simulink model "Kamerastabilisierung"  (R2026a)
settings: Solver=ode4  StopTime=SIM.Tend  FixedStep=SIM.Ts
values from neighbouring files (symbols this model uses):
  GEL = par_gelenk(Z1)    [start_model.m]
  HOE = par_hoehe(SIM, rauschen = STUFE >= 3)    [start_model.m]
  MONT = par_montage()    [start_model.m]
  REG = par_regler(SIM, Z1, MONT)    [start_model.m]
  SEN = par_sensor(SIM, rauschen = STUFE >= 3)    [start_model.m]
  SIM = par_sim("vorn")    [start_model.m]
undefined symbols (not defined in the file or in its folder): Z1
settings Model: NumberOfSteps=2  Creator=johannes  LastModifiedBy=johannes

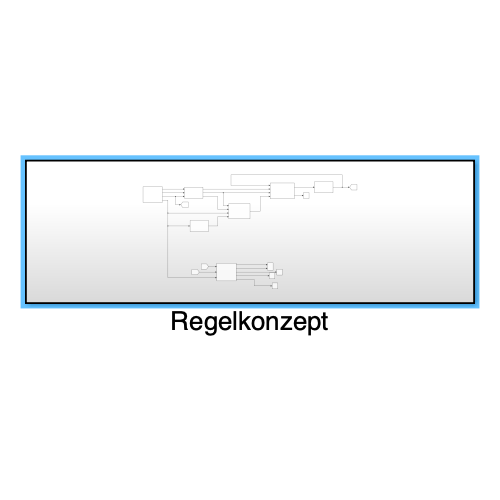
[thumbnail: Simulink's stored preview of the top-level diagram]
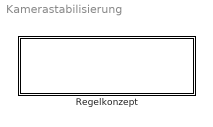
== system Kamerastabilisierung ==
  Regelkonzept : Subsystem

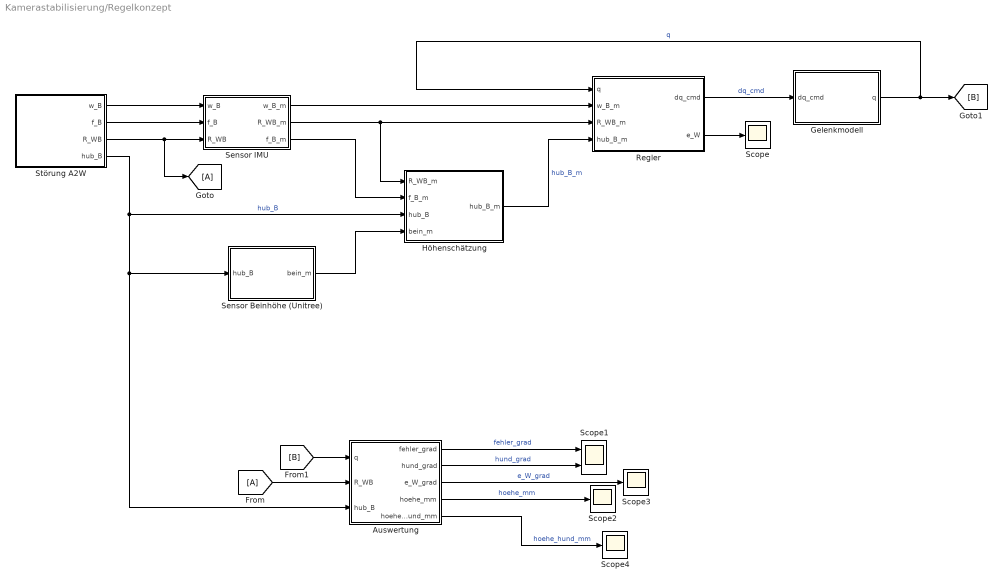
== system Kamerastabilisierung/Regelkonzept ==
  Auswertung : Subsystem
  From : From
  Gelenkmodell : Subsystem  Variant=on
  Goto : Goto
  Höhenschätzung : Subsystem  Variant=on
  Regler : Subsystem
  Scope{,2..4} (4 alike) : Scope
      Scope settings: ActiveDisplayYMinimum=-1  ActiveDisplayYMaximum=1  DataLoggingVariableName=ScopeData4
      Scope2 settings: ActiveDisplayYMinimum=-1  ActiveDisplayYMaximum=1
      Scope3 settings: ActiveDisplayYMinimum=-1  ActiveDisplayYMaximum=1  DataLoggingVariableName=ScopeData7
      Scope4 settings: ActiveDisplayYMinimum=-1  ActiveDisplayYMaximum=1  DataLoggingVariableName=ScopeData2
  Scope1 : Scope  NumInputPorts=2
      settings: ActiveDisplayYMinimum=-1  ActiveDisplayYMaximum=1
  Sensor Beinhöhe (Unitree) : Subsystem  Variant=on
  Sensor IMU : Subsystem  Variant=on
  Störung A2W : Subsystem
  wires:
  Störung A2W/3(R_WB) -> Goto/1, Sensor IMU/3(R_WB)
  Regler/2(e_W) -> Scope/1
  Auswertung/3(e_W_grad) -> Scope3/1  "e_W_grad"
  Auswertung/1(fehler_grad) -> Scope1/1  "fehler_grad"
  Auswertung/2(hund_grad) -> Scope1/2  "hund_grad"
  Störung A2W/1(w_B) -> Sensor IMU/1(w_B)
  Sensor IMU/1(w_B_m) -> Regler/2(w_B_m)
  Sensor IMU/2(R_WB_m) -> Regler/3(R_WB_m), Höhenschätzung/1(R_WB_m)
  Regler/1(dq_cmd) -> Gelenkmodell/1(dq_cmd)  "dq_cmd"
  Gelenkmodell/1(q) -> [B], Regler/1(q)  "q"
  Störung A2W/4(hub_B) -> Sensor Beinhöhe (Unitree)/1(hub_B), Auswertung/3(hub_B), Höhenschätzung/3(hub_B)  "hub_B"
  Auswertung/4(hoehe_mm) -> Scope2/1  "hoehe_mm"
  Auswertung/5(hoehe_hund_mm) -> Scope4/1  "hoehe_hund_mm"
  Störung A2W/2(f_B) -> Sensor IMU/2(f_B)
  Sensor IMU/3(f_B_m) -> Höhenschätzung/2(f_B_m)
  Höhenschätzung/1(hub_B_m) -> Regler/4(hub_B_m)  "hub_B_m"
  Sensor Beinhöhe (Unitree)/1(bein_m) -> Höhenschätzung/4(bein_m)
  From/1 -> Auswertung/2(R_WB)
  [B] -> Auswertung/1(q)

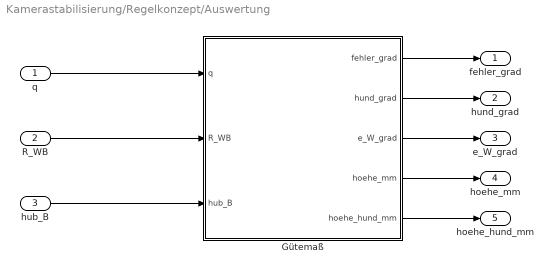
== system Kamerastabilisierung/Regelkonzept/Auswertung ==
  q : Inport
  R_WB : Inport  Port=2
  hub_B : Inport  Port=3
  Gütemaß : MATLAB Function  TreatAsAtomicUnit=on
  fehler_grad : Outport
  hund_grad : Outport  Port=2
  e_W_grad : Outport  Port=3
  hoehe_mm : Outport  Port=4
  hoehe_hund_mm : Outport  Port=5
  wires:
  Gütemaß/1(fehler_grad) -> fehler_grad/1
  Gütemaß/2(hund_grad) -> hund_grad/1
  Gütemaß/3(e_W_grad) -> e_W_grad/1
  hub_B/1 -> Gütemaß/3(hub_B)
  Gütemaß/4(hoehe_mm) -> hoehe_mm/1
  Gütemaß/5(hoehe_hund_mm) -> hoehe_hund_mm/1
  q/1 -> Gütemaß/1(q)
  R_WB/1 -> Gütemaß/2(R_WB)

== system Kamerastabilisierung/Regelkonzept/Gelenkmodell ==
  dq_cmd : Inport
  Ideal : Subsystem  VariantControl=STUFE == 1
  Realistisch : Subsystem  VariantControl=STUFE >= 2
  q : Outport

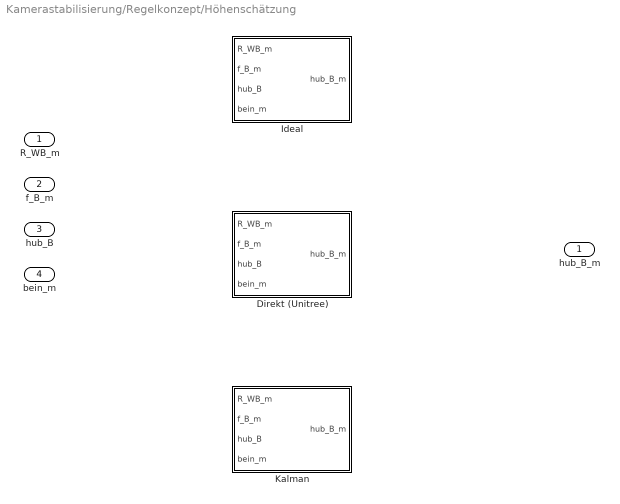
== system Kamerastabilisierung/Regelkonzept/Höhenschätzung ==
  R_WB_m : Inport
  f_B_m : Inport  Port=2
  hub_B : Inport  Port=3
  bein_m : Inport  Port=4
  Direkt (Unitree) : Subsystem  VariantControl=HOEHE_QUELLE == 2
  Ideal : Subsystem  VariantControl=HOEHE_QUELLE == 1
  Kalman : Subsystem  VariantControl=HOEHE_QUELLE == 3
  hub_B_m : Outport

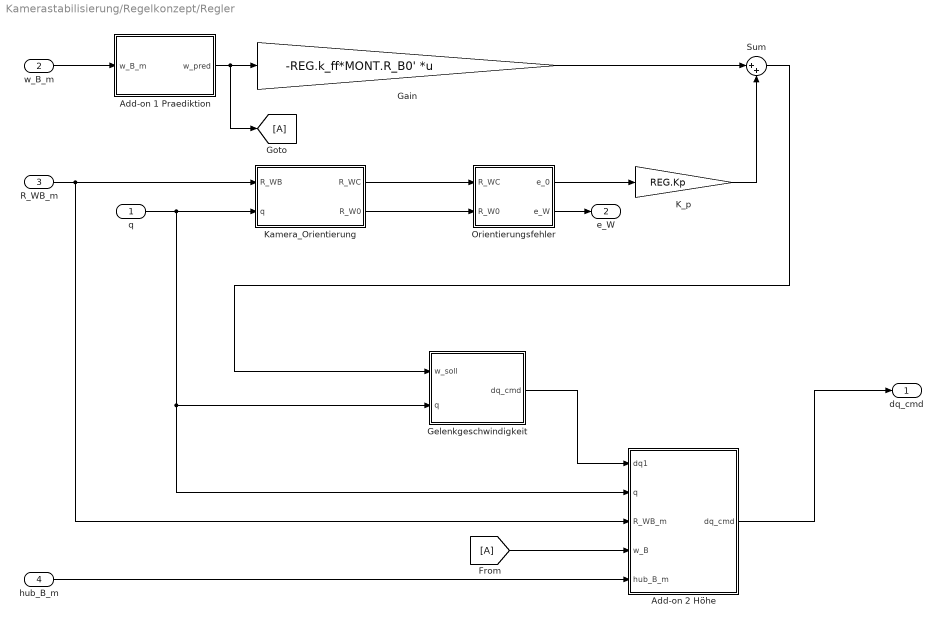
== system Kamerastabilisierung/Regelkonzept/Regler ==
  q : Inport
  w_B_m : Inport  Port=2
  R_WB_m : Inport  Port=3
  hub_B_m : Inport  Port=4
  Add-on 1 Praediktion : Subsystem  Variant=on
  Add-on 2 Höhe : Subsystem  Variant=on
  From : From
  Gain : Gain  Gain=-REG.k_ff*MONT.R_B0'  Multiplication=Matrix(K*u) (u vector)
  Gelenkgeschwindigkeit : MATLAB Function  TreatAsAtomicUnit=on
  Goto : Goto
  K_p : Gain  Gain=REG.Kp
  Kamera_Orientierung : MATLAB Function  TreatAsAtomicUnit=on
  Orientierungsfehler : MATLAB Function  TreatAsAtomicUnit=on
  Sum : Sum  Inputs=|++
  dq_cmd : Outport
  e_W : Outport  Port=2
  wires:
  R_WB_m/1 -> Add-on 2 Höhe/3(R_WB_m), Kamera_Orientierung/1(R_WB)
  Kamera_Orientierung/1(R_WC) -> Orientierungsfehler/1(R_WC)
  Kamera_Orientierung/2(R_W0) -> Orientierungsfehler/2(R_W0)
  Orientierungsfehler/1(e_0) -> K_p/1
  K_p/1 -> Sum/2
  Gain/1 -> Sum/1
  q/1 -> Add-on 2 Höhe/2(q), Gelenkgeschwindigkeit/2(q), Kamera_Orientierung/2(q)
  Sum/1 -> Gelenkgeschwindigkeit/1(w_soll)
  Orientierungsfehler/2(e_W) -> e_W/1
  w_B_m/1 -> Add-on 1 Praediktion/1(w_B_m)
  Add-on 1 Praediktion/1(w_pred) -> Goto/1, Gain/1
  Gelenkgeschwindigkeit/1(dq_cmd) -> Add-on 2 Höhe/1(dq1)
  hub_B_m/1 -> Add-on 2 Höhe/5(hub_B_m)
  Add-on 2 Höhe/1(dq_cmd) -> dq_cmd/1
  From/1 -> Add-on 2 Höhe/4(w_B)

== system Kamerastabilisierung/Regelkonzept/Sensor Beinhöhe (Unitree) ==
  hub_B : Inport
  Abgetastet : Subsystem  VariantControl=STUFE >= 2
  Ideal : Subsystem  VariantControl=STUFE == 1
  bein_m : Outport

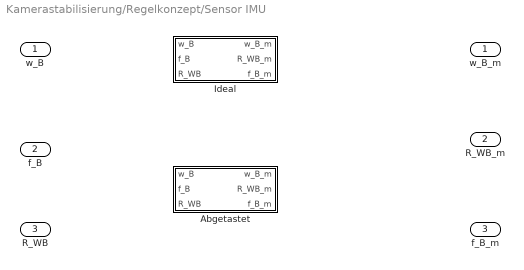
== system Kamerastabilisierung/Regelkonzept/Sensor IMU ==
  w_B : Inport
  f_B : Inport  Port=2
  R_WB : Inport  Port=3
  Abgetastet : Subsystem  VariantControl=STUFE >= 2
  Ideal : Subsystem  VariantControl=STUFE == 1
  w_B_m : Outport
  R_WB_m : Outport  Port=2
  f_B_m : Outport  Port=3

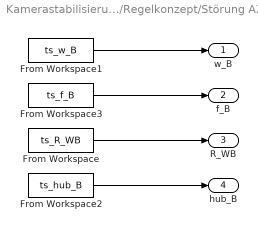
== system Kamerastabilisierung/Regelkonzept/Störung A2W ==
  From Workspace : FromWorkspace  VariableName=ts_R_WB  OutputAfterFinalValue=Holding final value
  From Workspace1 : FromWorkspace  VariableName=ts_w_B  OutputAfterFinalValue=Holding final value
  From Workspace2 : FromWorkspace  VariableName=ts_hub_B  OutputAfterFinalValue=Holding final value
  From Workspace3 : FromWorkspace  VariableName=ts_f_B  OutputAfterFinalValue=Holding final value
  w_B : Outport
  f_B : Outport  Port=2
  R_WB : Outport  Port=3
  hub_B : Outport  Port=4
  wires:
  From Workspace/1 -> R_WB/1
  From Workspace1/1 -> w_B/1
  From Workspace2/1 -> hub_B/1
  From Workspace3/1 -> f_B/1

== system Kamerastabilisierung/Regelkonzept/Gelenkmodell/Ideal ==
  dq_cmd : Inport
  Integrator : Integrator  InitialCondition=SIM.q0
  q : Outport
  wires:
  dq_cmd/1 -> Integrator/1
  Integrator/1 -> q/1

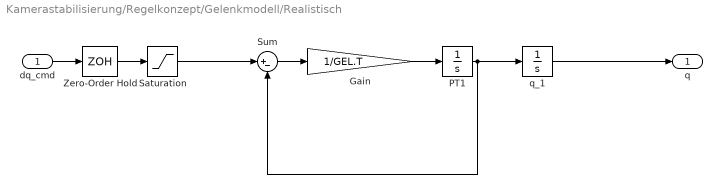
== system Kamerastabilisierung/Regelkonzept/Gelenkmodell/Realistisch ==
  dq_cmd : Inport
  Gain : Gain  Gain=1/GEL.T
  PT1 : Integrator
  Saturation : Saturate  UpperLimit=GEL.dq_max  LowerLimit=-GEL.dq_max
  Sum : Sum  Inputs=|+-
  Zero-Order Hold : ZeroOrderHold  SampleTime=SIM.Ts
  q_1 : Integrator  InitialCondition=SIM.q0  LimitOutput=on  UpperSaturationLimit=GEL.q_max  LowerSaturationLimit=GEL.q_min
  q : Outport
  wires:
  dq_cmd/1 -> Zero-Order Hold/1
  Zero-Order Hold/1 -> Saturation/1
  Saturation/1 -> Sum/1
  Sum/1 -> Gain/1
  Gain/1 -> PT1/1
  PT1/1 -> Sum/2, q_1/1
  q_1/1 -> q/1

== system Kamerastabilisierung/Regelkonzept/Höhenschätzung/Direkt (Unitree) ==
  R_WB_m : Inport
  f_B_m : Inport  Port=2
  hub_B : Inport  Port=3
  bein_m : Inport  Port=4
  Terminator : Terminator
  Terminator1 : Terminator
  Terminator2 : Terminator
  hub_B_m : Outport
  wires:
  f_B_m/1 -> Terminator/1
  R_WB_m/1 -> Terminator1/1
  bein_m/1 -> hub_B_m/1
  hub_B/1 -> Terminator2/1

== system Kamerastabilisierung/Regelkonzept/Höhenschätzung/Ideal ==
  R_WB_m : Inport
  f_B_m : Inport  Port=2
  hub_B : Inport  Port=3
  bein_m : Inport  Port=4
  Terminator : Terminator
  Terminator1 : Terminator
  Terminator2 : Terminator
  hub_B_m : Outport
  wires:
  hub_B/1 -> hub_B_m/1
  f_B_m/1 -> Terminator/1
  R_WB_m/1 -> Terminator1/1
  bein_m/1 -> Terminator2/1

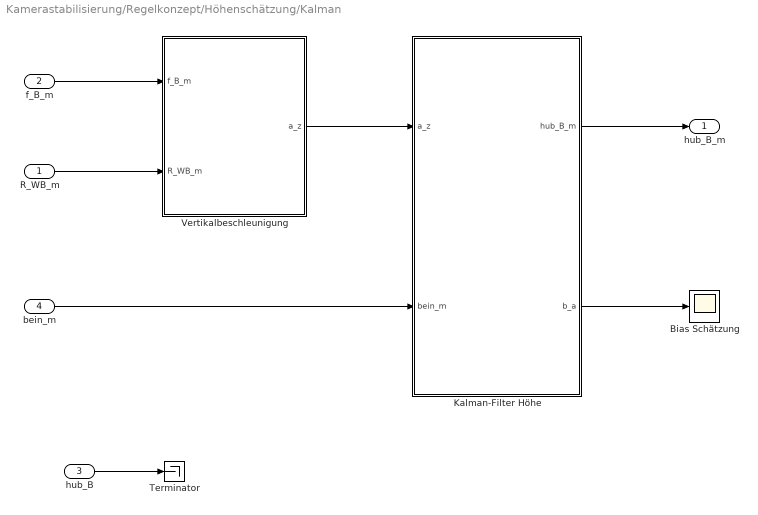
== system Kamerastabilisierung/Regelkonzept/Höhenschätzung/Kalman ==
  R_WB_m : Inport
  f_B_m : Inport  Port=2
  hub_B : Inport  Port=3
  bein_m : Inport  Port=4
  Bias Schätzung : Scope
      settings: DataLoggingVariableName=ScopeData5
  Kalman-Filter Höhe : MATLAB Function  TreatAsAtomicUnit=on
  Terminator : Terminator
  Vertikalbeschleunigung : MATLAB Function  TreatAsAtomicUnit=on
  hub_B_m : Outport
  wires:
  Vertikalbeschleunigung/1(a_z) -> Kalman-Filter Höhe/1(a_z)
  f_B_m/1 -> Vertikalbeschleunigung/1(f_B_m)
  R_WB_m/1 -> Vertikalbeschleunigung/2(R_WB_m)
  bein_m/1 -> Kalman-Filter Höhe/2(bein_m)
  hub_B/1 -> Terminator/1
  Kalman-Filter Höhe/1(hub_B_m) -> hub_B_m/1
  Kalman-Filter Höhe/2(b_a) -> Bias Schätzung/1

== system Kamerastabilisierung/Regelkonzept/Regler/Add-on 1 Praediktion ==
  w_B_m : Inport
  An : Subsystem  VariantControl=PRAEDIKTION == 1
  Aus : Subsystem  VariantControl=PRAEDIKTION == 0
  w_pred : Outport

== system Kamerastabilisierung/Regelkonzept/Regler/Add-on 2 Höhe ==
  dq1 : Inport
  q : Inport  Port=2
  R_WB_m : Inport  Port=3
  w_B : Inport  Port=4
  hub_B_m : Inport  Port=5
  An : Subsystem  VariantControl=HEAVE == 1
  Aus : Subsystem  VariantControl=HEAVE == 0
  dq_cmd : Outport

== system Kamerastabilisierung/Regelkonzept/Sensor Beinhöhe (Unitree)/Abgetastet ==
  hub_B : Inport
  Delay : Delay  DelayLength=HOE.N_bein
  Random Number : RandomNumber  Variance=HOE.var  Seed=HOE.seed  SampleTime=HOE.Ts
  Sum : Sum
  Zero-Order Hold : ZeroOrderHold  SampleTime=HOE.Ts
  bein_m : Outport
  wires:
  hub_B/1 -> Zero-Order Hold/1
  Delay/1 -> bein_m/1
  Sum/1 -> Delay/1
  Random Number/1 -> Sum/2
  Zero-Order Hold/1 -> Sum/1

== system Kamerastabilisierung/Regelkonzept/Sensor Beinhöhe (Unitree)/Ideal ==
  hub_B : Inport
  bein_m : Outport
  wires:
  hub_B/1 -> bein_m/1

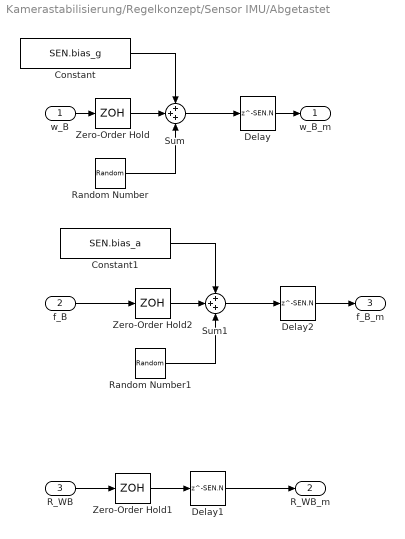
== system Kamerastabilisierung/Regelkonzept/Sensor IMU/Abgetastet ==
  w_B : Inport
  f_B : Inport  Port=2
  R_WB : Inport  Port=3
  Constant : Constant  Value=SEN.bias_g  VectorParams1D=off
  Constant1 : Constant  Value=SEN.bias_a  VectorParams1D=off
  Delay : Delay  DelayLength=SEN.N
  Delay1 : Delay  DelayLength=SEN.N  InitialCondition=SEN.R0
  Delay2 : Delay  DelayLength=SEN.N  InitialCondition=SEN.f0
  Random Number : RandomNumber  Mean=zeros(3,1)  Variance=SEN.var_g  Seed=SEN.seed_g  SampleTime=SIM.Ts  VectorParams1D=off
  Random Number1 : RandomNumber  Mean=zeros(3,1)  Variance=SEN.var_a  Seed=SEN.seed_a  SampleTime=SIM.Ts  VectorParams1D=off
  Sum : Sum  Inputs=+++
  Sum1 : Sum  Inputs=+++
  Zero-Order Hold : ZeroOrderHold  SampleTime=SIM.Ts
  Zero-Order Hold1 : ZeroOrderHold  SampleTime=SIM.Ts
  Zero-Order Hold2 : ZeroOrderHold  SampleTime=SIM.Ts
  w_B_m : Outport
  R_WB_m : Outport  Port=2
  f_B_m : Outport  Port=3
  wires:
  w_B/1 -> Zero-Order Hold/1
  Delay/1 -> w_B_m/1
  Zero-Order Hold1/1 -> Delay1/1
  R_WB/1 -> Zero-Order Hold1/1
  Delay1/1 -> R_WB_m/1
  Zero-Order Hold/1 -> Sum/2
  Sum/1 -> Delay/1
  Constant/1 -> Sum/1
  Random Number/1 -> Sum/3
  f_B/1 -> Zero-Order Hold2/1
  Random Number1/1 -> Sum1/3
  Zero-Order Hold2/1 -> Sum1/2
  Delay2/1 -> f_B_m/1
  Sum1/1 -> Delay2/1
  Constant1/1 -> Sum1/1

== system Kamerastabilisierung/Regelkonzept/Sensor IMU/Ideal ==
  w_B : Inport
  f_B : Inport  Port=2
  R_WB : Inport  Port=3
  w_B_m : Outport
  R_WB_m : Outport  Port=2
  f_B_m : Outport  Port=3
  wires:
  R_WB/1 -> R_WB_m/1
  w_B/1 -> w_B_m/1
  f_B/1 -> f_B_m/1

== system Kamerastabilisierung/Regelkonzept/Regler/Add-on 1 Praediktion/An ==
  note: „Add-on 1 nach Woolfrey et al. 2021, Gl. (7): ŷ(t) = Σ αᵢ·y(t−i). αᵢ per Kleinste Quadrate über die letzten M = 250 Gyro-Werte, Vorhersage um h = τ_eff/T_s = 16 Schritte (31 ms).“
  w_B_m : Inport
  AR-Vorhersage : MATLAB Function  TreatAsAtomicUnit=on
  Messfenster (letzte M Werte) : MATLAB Function  TreatAsAtomicUnit=on
  Switch : Switch  Criteria=u2 > Threshold  Threshold=0.5  SaturateOnIntegerOverflow=off  InputSameDT=off
  w_pred : Outport
  wires:
  AR-Vorhersage/1(w_ar) -> Switch/1
  Messfenster (letzte M Werte)/2(voll) -> Switch/2
  w_B_m/1 -> Messfenster (letzte M Werte)/1(w_m), Switch/3
  Switch/1 -> w_pred/1
  Messfenster (letzte M Werte)/1(fenster) -> AR-Vorhersage/1(fenster)

== system Kamerastabilisierung/Regelkonzept/Regler/Add-on 1 Praediktion/Aus ==
  w_B_m : Inport
  w_pred : Outport
  wires:
  w_B_m/1 -> w_pred/1

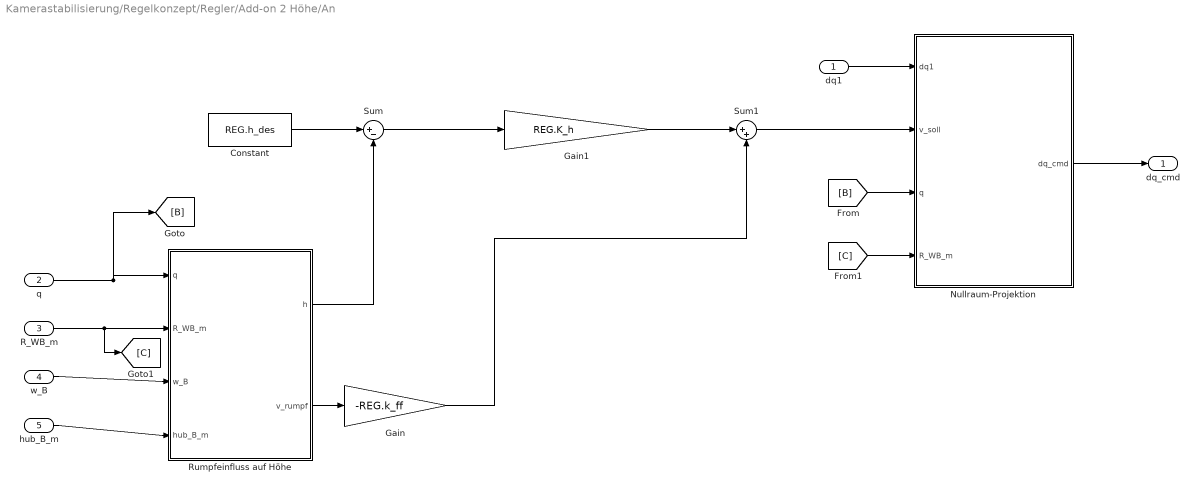
== system Kamerastabilisierung/Regelkonzept/Regler/Add-on 2 Höhe/An ==
  dq1 : Inport
  q : Inport  Port=2
  R_WB_m : Inport  Port=3
  w_B : Inport  Port=4
  hub_B_m : Inport  Port=5
  Constant : Constant  Value=REG.h_des
  Gain : Gain  Gain=-REG.k_ff
  Gain1 : Gain  Gain=REG.K_h
  Nullraum-Projektion : MATLAB Function  TreatAsAtomicUnit=on
  Rumpfeinfluss auf Höhe : MATLAB Function  TreatAsAtomicUnit=on
  Sum : Sum  Inputs=|+-
  Sum1 : Sum  Inputs=|++
  dq_cmd : Outport
  wires:
  q/1 -> [B], Rumpfeinfluss auf Höhe/1(q)
  R_WB_m/1 -> [C], Rumpfeinfluss auf Höhe/2(R_WB_m)
  w_B/1 -> Rumpfeinfluss auf Höhe/3(w_B)
  hub_B_m/1 -> Rumpfeinfluss auf Höhe/4(hub_B_m)
  Rumpfeinfluss auf Höhe/2(v_rumpf) -> Gain/1
  Constant/1 -> Sum/1
  Rumpfeinfluss auf Höhe/1(h) -> Sum/2
  Sum/1 -> Gain1/1
  Gain1/1 -> Sum1/1
  Gain/1 -> Sum1/2
  Sum1/1 -> Nullraum-Projektion/2(v_soll)
  dq1/1 -> Nullraum-Projektion/1(dq1)
  [B] -> Nullraum-Projektion/3(q)
  [C] -> Nullraum-Projektion/4(R_WB_m)
  Nullraum-Projektion/1(dq_cmd) -> dq_cmd/1

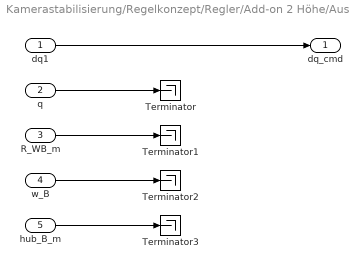
== system Kamerastabilisierung/Regelkonzept/Regler/Add-on 2 Höhe/Aus ==
  dq1 : Inport
  q : Inport  Port=2
  R_WB_m : Inport  Port=3
  w_B : Inport  Port=4
  hub_B_m : Inport  Port=5
  Terminator{,1..3} (4 alike) : Terminator
  dq_cmd : Outport
  wires:
  dq1/1 -> dq_cmd/1
  q/1 -> Terminator/1
  R_WB_m/1 -> Terminator1/1
  w_B/1 -> Terminator2/1
  hub_B_m/1 -> Terminator3/1

== matlab function Kamerastabilisierung/Regelkonzept/Höhenschätzung/Kalman/Vertikalbeschleunigung ==
  data: f_B_m input; a_z output; R_WB_m input; KAL parameter
  function a_z = fcn(f_B_m, R_WB_m, KAL)
  % Spezifische Kraft ins Weltsystem drehen und Schwerkraft abziehen (Meng Gl. 43 umgestellt)
  a_z = [0 0 1] * R_WB_m * f_B_m(:) - KAL.g;
  end

== matlab function Kamerastabilisierung/Regelkonzept/Höhenschätzung/Kalman/Kalman-Filter Höhe ==
  settings: updateMethod=DISCRETE  sampleTime=KAL.Ts
  data: a_z input; hub_B_m output; bein_m input; b_a output; KAL parameter
  function [hub_B_m, b_a] = fcn(a_z, bein_m, KAL)
  % Zustand [z; dz; b_a] bleibt zwischen den Abtastschritten erhalten (persistent)
  persistent x P ubuf
  if isempty(x)
      x    = zeros(3, 1);
      P    = KAL.P0;
      ubuf = zeros(1, KAL.d + 2);
  end
  [x, P, ubuf, hub_B_m] = kalman_hoehe(x, P, ubuf, a_z, bein_m, KAL);
  b_a = x(3);                 % geschätzter Bias (zum Anschauen im Scope)
  end

== matlab function Kamerastabilisierung/Regelkonzept/Regler/Add-on 1 Praediktion/An/Messfenster (letzte M Werte) ==
  settings: updateMethod=DISCRETE  sampleTime=SIM.Ts
  data: w_m input; fenster output; PRAED parameter; voll output
function [fenster, voll] = fcn(w_m, PRAED)
% Merkt sich die letzten PRAED.M Gyro-Messwerte.
% fenster: Zeile = Zeitpunkt (ältester oben, neuester unten), Spalte = Achse
% voll:    1, sobald M Werte gesammelt sind
persistent puffer anzahl
if isempty(puffer)
    puffer = zeros(PRAED.M, 3);
    anzahl = 0;
end
puffer  = [puffer(2:end, :); w_m(:).'];
anzahl  = min(anzahl + 1, PRAED.M);
fenster = puffer;
voll    = double(anzahl == PRAED.M);
end

== matlab function Kamerastabilisierung/Regelkonzept/Regler/Add-on 2 Höhe/An/Rumpfeinfluss auf Höhe ==
  data: q input; h output; R_WB_m input; w_B input; hub_B_m input; v_rumpf output; Z1 parameter; MONT parameter
  function [h, v_rumpf] = fcn(q, R_WB_m, w_B, hub_B_m, Z1, MONT)
  % Höhe des Endeffektors und Vertikalgeschwindigkeit, die der Rumpf allein verursacht
  [h, v_rumpf] = hoehe_aufschaltung(q, R_WB_m, w_B, hub_B_m(1), hub_B_m(2), Z1, MONT);
  end

== matlab function Kamerastabilisierung/Regelkonzept/Regler/Add-on 1 Praediktion/An/AR-Vorhersage ==
  settings: updateMethod=DISCRETE  sampleTime=SIM.Ts
  data: fenster input; w_ar output; PRAED parameter
function w_ar = fcn(fenster, PRAED)
% Quelle: Woolfrey et al. 2021, Abschnitt III, Gl. (7)
% Je Achse: AR(p)-Gewichte per Kleinste Quadrate aus dem Fenster schätzen,
% dann um h Schritte (= tau_eff) vorhersagen.
w_ar = zeros(3, 1);
for a = 1:3
    w_ar(a) = ar_praediktion(fenster(:, a), PRAED.p, PRAED.h, PRAED.mu);
end
end

== matlab function Kamerastabilisierung/Regelkonzept/Regler/Add-on 2 Höhe/An/Nullraum-Projektion ==
  data: dq1 input; dq_cmd output; v_soll input; q input; R_WB_m input; Z1 parameter; MONT parameter; REG parameter
  function dq_cmd = fcn(dq1, v_soll, q, R_WB_m, Z1, MONT, REG)
  % Höhe nur im Nullraum der Orientierung -> Orientierung hat Vorrang
  dq_cmd = nullraum_hoehe(dq1, v_soll, q, R_WB_m, Z1, MONT, REG.lambda);
  end

== matlab function Kamerastabilisierung/Regelkonzept/Auswertung/Gütemaß ==
  data: q input; R_WB input; fehler_grad output; hub_B input; hund_grad output; e_W_grad output; Z1 parameter; REG parameter; MONT parameter; hoehe_mm output; hoehe_hund_mm output
function [fehler_grad, hund_grad, e_W_grad, hoehe_mm, hoehe_hund_mm] = fcn(q, R_WB, hub_B, Z1, REG, MONT)
% Hauptgütemaß: Orientierungsfehler der Kamera im Weltsystem in Grad,
% berechnet mit der WAHREN Rumpflage.
R_WC = kamera_orientierung(q, R_WB, Z1, MONT);
e_W  = rot_log(REG.R_WC_des * R_WC');
fehler_grad = norm(e_W) * 180/pi;
e_W_grad    = e_W * 180/pi;

% Vergleich "ohne Stabilisierung": Fehler = Drehwinkel des Rumpfes seit Start
hund_grad = norm(rot_log(R_WB)) * 180/pi;

% Add-on 2: Höhenfehler des Endeffektors gegenüber der Sollhöhe [mm]
% mit der WAHREN Rumpfbewegung (hub_B = [z_B; dz_B])
hoehe_mm      = 1000 * (ee_hoehe(q,      R_WB, hub_B(1), Z1, MONT) - REG.h_des);
% Vergleich "ohne Stabilisierung": Arm steif in der Grundpose
hoehe_hund_mm = 1000 * (ee_hoehe(REG.q0, R_WB, hub_B(1), Z1, MONT) - REG.h_des);
end

== matlab function Kamerastabilisierung/Regelkonzept/Regler/Gelenkgeschwindigkeit ==
  data: w_soll input; q input; dq_cmd output; Z1 parameter; MONT parameter; REG parameter
function dq_cmd = fcn(w_soll, q, Z1, MONT, REG)
% dq_cmd = J_w#(q) * w_soll   (gedämpfte Pseudoinverse, Buss 2004)
J      = z1_jacobian(q, Z1, MONT.T_6C);
J_w    = J(4:6, :);
dq_cmd = dls_pinv(J_w, REG.lambda) * w_soll;
end

== matlab function Kamerastabilisierung/Regelkonzept/Regler/Kamera_Orientierung ==
  data: R_WB input; q input; R_WC output; R_W0 output; Z1 parameter; MONT parameter
function [R_WC, R_W0] = fcn(R_WB, q, Z1, MONT)
% KAMERA_ORIENTIERUNG (Simulink-Block im Regler)
% Orientierung der Kamera im Weltsystem aus Rumpflage und Gelenkwinkeln:
%   R_W0 = R_WB * R_B0              Basis des Z1 im Weltsystem
%   R_WC = R_W0 * R_0C(q)           Kamera im Weltsystem
% Die Rechnung steckt in der getesteten Funktion kamera_orientierung.m,
% damit Regler und Auswertung garantiert dasselbe rechnen.
[R_WC, R_W0] = kamera_orientierung(q, R_WB, Z1, MONT);
end

== matlab function Kamerastabilisierung/Regelkonzept/Regler/Orientierungsfehler ==
  data: R_WC input; e_0 output; R_W0 input; e_W output; REG parameter
function [e_0, e_W] = fcn(R_WC, R_W0, REG)
% Fehler als Achse*Winkel: e_W im Weltsystem, e_0 im Basisframe 0
[e_0, e_W] = orient_fehler(R_WC, REG.R_WC_des, R_W0);
end
